simulink model "DC_Pool_Capacity_Fault_20261023_SK"  (R2026a)
settings: Solver=FixedStepDiscrete  StopTime=604800  FixedStep=300
undefined symbols (not defined in the file or in its folder): cl_cop_pool, cl_mode, cl_params, cl_source_temp
settings Model: Creator=Lysda  LastModifiedBy=Lysda

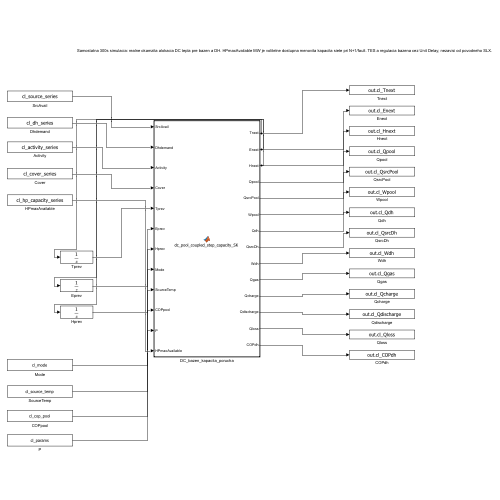
[thumbnail: Simulink's stored preview of the top-level diagram]
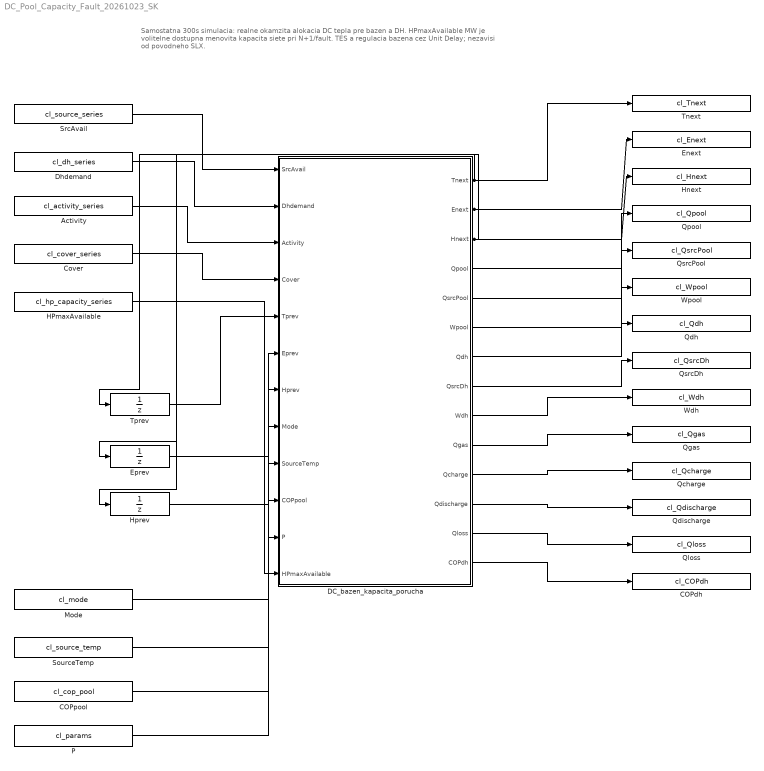
== system DC_Pool_Capacity_Fault_20261023_SK ==
  note: Samostatna 300s simulacia: realne okamzita alokacia DC tepla pre bazen a DH. HPmaxAvailable MW je volitelne dostupna menovita kapacita siete pri N+1/fault. TES a regulacia bazena cez Unit Delay; nezavisi od povodneho SLX.
  Activity : FromWorkspace  VariableName=cl_activity_series
  COPdh : ToWorkspace  VariableName=cl_COPdh  SaveFormat=Timeseries  SampleTime=-1
  COPpool : Constant  Value=cl_cop_pool
  Cover : FromWorkspace  VariableName=cl_cover_series
  DC_bazen_kapacita_porucha : MATLAB Function  TreatAsAtomicUnit=on
  Dhdemand : FromWorkspace  VariableName=cl_dh_series
  Enext : ToWorkspace  VariableName=cl_Enext  SaveFormat=Timeseries  SampleTime=-1
  Eprev : UnitDelay  SampleTime=300
  HPmaxAvailable : FromWorkspace  VariableName=cl_hp_capacity_series
  Hnext : ToWorkspace  VariableName=cl_Hnext  SaveFormat=Timeseries  SampleTime=-1
  Hprev : UnitDelay  InitialCondition=1  SampleTime=300
  Mode : Constant  Value=cl_mode
  P : Constant  Value=cl_params
  Qcharge : ToWorkspace  VariableName=cl_Qcharge  SaveFormat=Timeseries  SampleTime=-1
  Qdh : ToWorkspace  VariableName=cl_Qdh  SaveFormat=Timeseries  SampleTime=-1
  Qdischarge : ToWorkspace  VariableName=cl_Qdischarge  SaveFormat=Timeseries  SampleTime=-1
  Qgas : ToWorkspace  VariableName=cl_Qgas  SaveFormat=Timeseries  SampleTime=-1
  Qloss : ToWorkspace  VariableName=cl_Qloss  SaveFormat=Timeseries  SampleTime=-1
  Qpool : ToWorkspace  VariableName=cl_Qpool  SaveFormat=Timeseries  SampleTime=-1
  QsrcDh : ToWorkspace  VariableName=cl_QsrcDh  SaveFormat=Timeseries  SampleTime=-1
  QsrcPool : ToWorkspace  VariableName=cl_QsrcPool  SaveFormat=Timeseries  SampleTime=-1
  SourceTemp : Constant  Value=cl_source_temp
  SrcAvail : FromWorkspace  VariableName=cl_source_series
  Tnext : ToWorkspace  VariableName=cl_Tnext  SaveFormat=Timeseries  SampleTime=-1
  Tprev : UnitDelay  InitialCondition=16  SampleTime=300
  Wdh : ToWorkspace  VariableName=cl_Wdh  SaveFormat=Timeseries  SampleTime=-1
  Wpool : ToWorkspace  VariableName=cl_Wpool  SaveFormat=Timeseries  SampleTime=-1
  wires:
  SrcAvail/1 -> DC_bazen_kapacita_porucha/1(SrcAvail)
  Dhdemand/1 -> DC_bazen_kapacita_porucha/2(Dhdemand)
  Activity/1 -> DC_bazen_kapacita_porucha/3(Activity)
  Cover/1 -> DC_bazen_kapacita_porucha/4(Cover)
  Tprev/1 -> DC_bazen_kapacita_porucha/5(Tprev)
  Eprev/1 -> DC_bazen_kapacita_porucha/6(Eprev)
  Hprev/1 -> DC_bazen_kapacita_porucha/7(Hprev)
  Mode/1 -> DC_bazen_kapacita_porucha/8(Mode)
  SourceTemp/1 -> DC_bazen_kapacita_porucha/9(SourceTemp)
  COPpool/1 -> DC_bazen_kapacita_porucha/10(COPpool)
  P/1 -> DC_bazen_kapacita_porucha/11(P)
  HPmaxAvailable/1 -> DC_bazen_kapacita_porucha/12(HPmaxAvailable)
  DC_bazen_kapacita_porucha/1(Tnext) -> Tnext/1, Tprev/1
  DC_bazen_kapacita_porucha/2(Enext) -> Enext/1, Eprev/1
  DC_bazen_kapacita_porucha/3(Hnext) -> Hnext/1, Hprev/1
  DC_bazen_kapacita_porucha/4(Qpool) -> Qpool/1
  DC_bazen_kapacita_porucha/5(QsrcPool) -> QsrcPool/1
  DC_bazen_kapacita_porucha/6(Wpool) -> Wpool/1
  DC_bazen_kapacita_porucha/7(Qdh) -> Qdh/1
  DC_bazen_kapacita_porucha/8(QsrcDh) -> QsrcDh/1
  DC_bazen_kapacita_porucha/9(Wdh) -> Wdh/1
  DC_bazen_kapacita_porucha/10(Qgas) -> Qgas/1
  DC_bazen_kapacita_porucha/11(Qcharge) -> Qcharge/1
  DC_bazen_kapacita_porucha/12(Qdischarge) -> Qdischarge/1
  DC_bazen_kapacita_porucha/13(Qloss) -> Qloss/1
  DC_bazen_kapacita_porucha/14(COPdh) -> COPdh/1

== matlab function DC_Pool_Capacity_Fault_20261023_SK/DC_bazen_kapacita_porucha ==
  data: SrcAvail input; Tnext output; Dhdemand input; Activity input; Cover input; Tprev input; Eprev input; Hprev input; Mode input; SourceTemp input; COPpool input; P input; HPmaxAvailable input; Enext output; Hnext output; Qpool output; QsrcPool output; Wpool output; Qdh output; QsrcDh output; Wdh output; Qgas output; Qcharge output; Qdischarge output; Qloss output; COPdh output
function [Tnext,Enext,Hnext,Qpool,QsrcPool,Wpool,Qdh,QsrcDh,Wdh,Qgas,Qcharge,Qdischarge,Qloss,COPdh] = ...
 dc_pool_coupled_step_capacity_SK(SrcAvail,Dhdemand,Activity,Cover,Tprev,Eprev,Hprev,Mode,SourceTemp,COPpool,P,HPmaxAvailable)
%#codegen
% Capacity + failover study. OWN copy, previous Simulink source unmodified.
% All thermal powers are MW. HPmaxAvailable [MW useful] 0..12.
Cp=P(1); A=P(2); UA=P(3); MaxPoolW=P(4)*1e6;
Ton=P(5); Toff=P(6); Tmax=P(7); dt=P(8);
etaC=P(9); Tdh=P(10); MaxDH=P(11);
TEScap=P(12); QchargeMax=P(13); QdischargeMax=P(14);
etaCharge=P(15); etaDischarge=P(16); leakPerHour=P(17);
COPmin=P(18); COPmax=P(19);
QlossW=0;QpoolW=0;QsourcePoolW=0;WpoolW=0;Hnext=Hprev;
if Mode>0.5
  pv=0.61094*exp(17.625*Tprev/(Tprev+243.04));
  pa=0.6*0.61094*exp(17.625*29/(29+243.04));
  mEvap=max(0,4e-5*A*(pv-pa)*Activity*(1-0.90*Cover));
  qEvap=mEvap*2440000;
  qConv=3*A*(Tprev-29)*(1-0.75*Cover);
  qRad=0.95*5.670374419e-8*A*((Tprev+273.15)^4-(27+273.15)^4)*(1-0.75*Cover);
  qGround=UA*(Tprev-20);
  qMakeup=mEvap*4182*(Tprev-15);
  QlossW=qEvap+qConv+qRad+qGround+qMakeup+2000;
  if Tprev<=Ton,Hnext=1;end
  if Tprev>=Toff,Hnext=0;end
  heatAllowed=(Mode>1.5 || SourceTemp>=Tprev+3);
  if Hnext>0.5 && heatAllowed
    qSafe=max(0,(Tmax-Tprev)*Cp/dt+QlossW);
    QpoolW=min(MaxPoolW,qSafe);
    if Mode>1.5
      qPoolCap=max(0,SrcAvail*1e6)*COPpool/(COPpool-1);
      QpoolW=min(QpoolW,qPoolCap);
      WpoolW=QpoolW/COPpool;
      QsourcePoolW=QpoolW-WpoolW;
    else
      QpoolW=min(QpoolW,max(0,SrcAvail*1e6));
      QsourcePoolW=QpoolW;
    end
  end
end
Tnext=Tprev+(QpoolW-QlossW)*dt/Cp;
Qpool=QpoolW/1e6;QsrcPool=QsourcePoolW/1e6;
Wpool=WpoolW/1e6;Qloss=QlossW/1e6;
remainder=max(0,SrcAvail-QsrcPool);
TdhK=Tdh+273.15;TsourceK=SourceTemp+273.15;
lift=max(1,TdhK-TsourceK);
COPdh=min(COPmax,max(COPmin,etaC*TdhK/lift));
% Live nameplate cap/failure enters on same sample and physically reallocates
% missing heat to TES/gas. Not a substitute for independent IT cooling.
possible=min(min(MaxDH,max(0,HPmaxAvailable)),remainder*COPdh/(COPdh-1));
Eavailable=Eprev*max(0,1-leakPerHour*dt/3600);
Qdh=0;Qgas=0;Qcharge=0;Qdischarge=0;
if possible>=Dhdemand
    Qdh=Dhdemand;
    if TEScap>0
        room=max(0,TEScap-Eavailable);
        Qcharge=min(min(possible-Dhdemand,QchargeMax),room/(etaCharge*dt/3600));
    end
    Qdh=Qdh+Qcharge;
    Enext=Eavailable+etaCharge*Qcharge*dt/3600;
else
    Qdh=possible;
    deficit=max(0,Dhdemand-possible);
    if TEScap>0
        Qdischarge=min(min(deficit,QdischargeMax),Eavailable*etaDischarge/(dt/3600));
    end
    Enext=max(0,Eavailable-Qdischarge*dt/3600/etaDischarge);
    Qgas=max(0,deficit-Qdischarge);
end
Wdh=Qdh/COPdh;
QsrcDh=Qdh-Wdh;
end
